simulink model "laba8"  (R2023b)
settings: Solver=VariableStepAuto  StartTime=0.0  StopTime=10.0  RelTol=1e-3
settings Model: Creator=user  LastModifiedBy=user

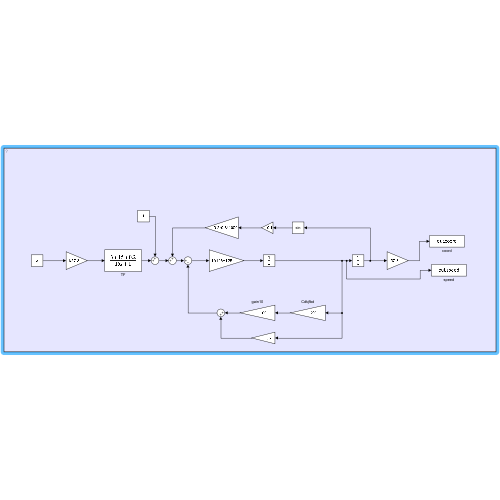
[thumbnail: Simulink's stored preview of the top-level diagram]
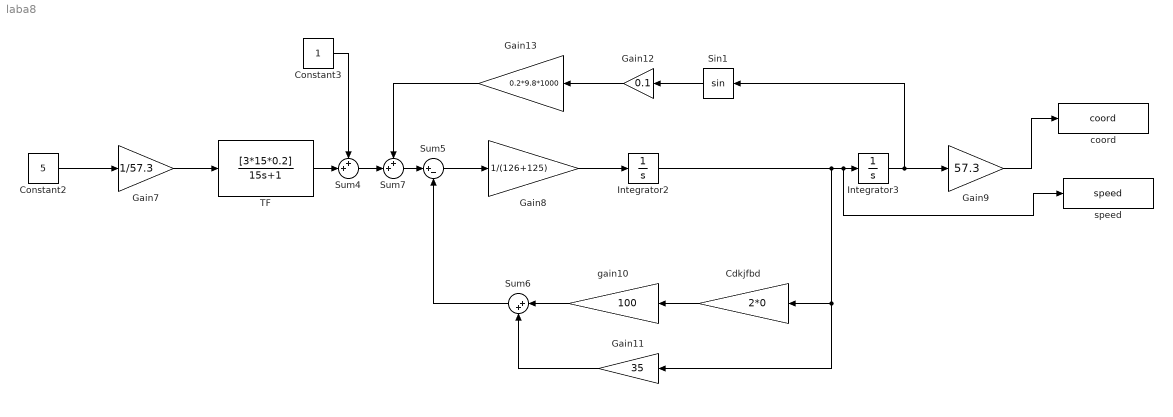
== system laba8 ==
  Cdkjfbd : Gain  Gain=2*0
  Constant2 : Constant  Value=5
  Constant3 : Constant
  Gain11 : Gain  Gain=35
  Gain12 : Gain  Gain=0.1
  Gain13 : Gain  Gain=0.2*9.8*1000
  Gain7 : Gain  Gain=1/57.3
  Gain8 : Gain  Gain=1/(126+125)
  Gain9 : Gain  Gain=57.3
  Integrator2 : Integrator
  Integrator3 : Integrator
  Sin1 : Trigonometry
  Sum4 : Sum  Inputs=++|
  Sum5 : Sum  Inputs=|+-
  Sum6 : Sum  Inputs=|++
  Sum7 : Sum  Inputs=++|
  TF : TransferFcn  Numerator=[3*15*0.2]  Denominator=[15 1]
  coord : ToWorkspace  VariableName=coord  SaveFormat=Timeseries  SampleTime=-1
  gain10 : Gain  Gain=100
  speed : ToWorkspace  VariableName=speed  SaveFormat=Timeseries  SampleTime=-1
  wires:
  Integrator2/1 -> speed/1, Integrator3/1, Gain11/1, Cdkjfbd/1
  Integrator3/1 -> Sin1/1, Gain9/1
  Sum4/1 -> Sum7/2
  TF/1 -> Sum4/2
  Gain11/1 -> Sum6/2
  Sum7/1 -> Sum5/1
  Constant2/1 -> Gain7/1
  Constant3/1 -> Sum4/1
  Gain7/1 -> TF/1
  Sin1/1 -> Gain12/1
  gain10/1 -> Sum6/1
  Sum5/1 -> Gain8/1
  Gain12/1 -> Gain13/1
  Gain8/1 -> Integrator2/1
  Gain13/1 -> Sum7/1
  Sum6/1 -> Sum5/2
  Gain9/1 -> coord/1
  Cdkjfbd/1 -> gain10/1
